simulink model "Resorte_Amoritguador"  (R2025a)
settings: Solver=VariableStepAuto  StartTime=0.0  StopTime=100  RelTol=1e-8
undefined symbols (not defined in the file): gamma, k, m
libraries: fl_lib x6, nesl_utility x3, sdl_lib x1
settings Model: Creator=LAPTOP  LastModifiedBy=LAPTOP

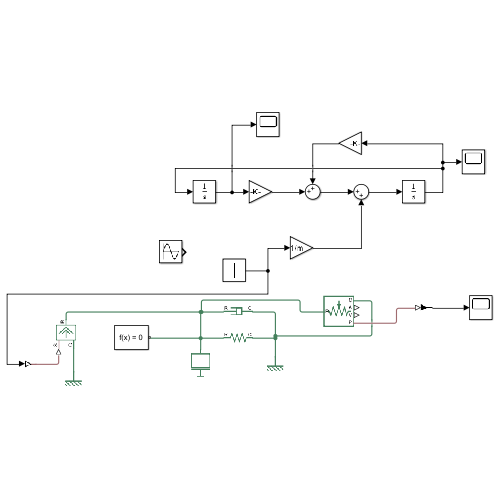
[thumbnail: Simulink's stored preview of the top-level diagram]
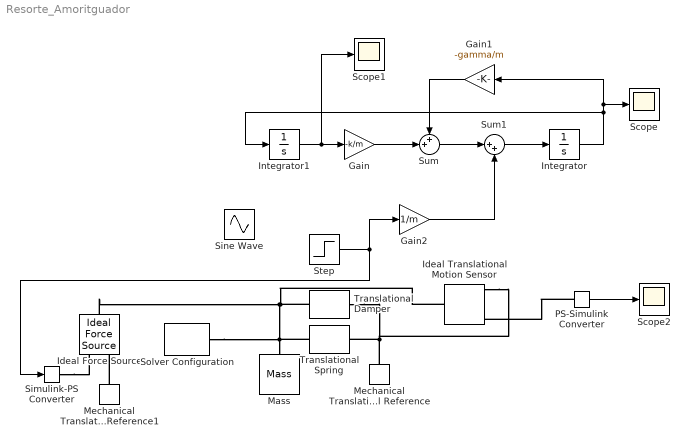
== system Resorte_Amoritguador ==
  Gain : Gain  Gain=-k/m
  Gain1 : Gain  Gain=-gamma/m
  Gain2 : Gain  Gain=1/m
  Ideal Force Source : fl_lib/Mechanical/Mechanical Sources/Ideal Force Source
  Ideal Translational Motion Sensor : fl_lib/Mechanical/Mechanical Sensors/Ideal Translational Motion Sensor  reference=foundation.enum.MeasurementReference.difference  acceleration_port=true  velocity_port=true  position_port=true  offset=0 m
      settings: InternalSimscapePortConfiguration="{\"Bottom\":[],\"Left\":[{\"id\":\"R\",\"label\":\"R\",\"type\":\"foundation.mechanical.translational.translational\"}],\"Right\":[{\"id\":\"C\",\"label\":\"C\",\"type\":\"foundation.mechanical.translational.translational\"},{\"id\":\"A\",\"label\":\"A\",\"type\":\"output\"},{\"id\":\"V\",\"label\":\"V\",\"type\":\"output\"},{\"id\":\"P\",\"label\":\"P\",\"type\":\"output\"}],\"Top\":[]}"
  Integrator : Integrator  InitialCondition=1
  Integrator1 : Integrator
  Mass : fl_lib/Mechanical/Translational Elements/Mass  mass=1 kg  num_ports=foundation.enum.numPorts2.one  v_specify=off  v_priority=High  v=0 m/s  v_nominal_specify=off  v_nominal_value=1  v_nominal_unit=m/s  f_specify=off  f_priority=None  f=0 N  f_nominal_specify=off  f_nominal_value=1  f_nominal_unit=N
  Mechanical Translational Reference : fl_lib/Mechanical/Translational Elements/Mechanical Translational Reference
  Mechanical Translational Reference1 : fl_lib/Mechanical/Translational Elements/Mechanical Translational Reference
  PS-Simulink Converter : nesl_utility/PS-Simulink Converter  PhysicalDomain=network_engine_domain  SubClassName=ps_output  LeftPortType=input  RightPortType=output  PseudoPeriodic=off  Frequencies=[]  VectorFormat=inherit  Unit=mm  AffineConversion=off
  Scope : Scope
      settings: ActiveDisplayYMinimum=-0.99836640803598919  ActiveDisplayYMaximum=1.2220407120039987
  Scope1 : Scope
      settings: ActiveDisplayYMinimum=-0.45113896464501263  ActiveDisplayYMaximum=0.66712367458581923
  Scope2 : Scope
      settings: ActiveDisplayYMinimum=-0.14841442149301454  ActiveDisplayYMaximum=1.1640855785069844  DataLoggingVariableName=ScopeData2
  Simulink-PS Converter : nesl_utility/Simulink-PS Converter  PhysicalDomain=network_engine_domain  SubClassName=ps_input  LeftPortType=input  RightPortType=output  PseudoPeriodic=off  Frequencies=[]  NoiseDistribution=none  NoiseParameters=[]  Unit=1  AffineConversion=off  FilteringAndDerivatives=provide  SimscapeFilterOrder=1  InputFilterTimeConstant=0.001  UdotUserProvided=0
  Sine Wave : Sin  SampleTime=0
  Solver Configuration : nesl_utility/Solver Configuration  PhysicalDomain=network_engine_domain  SubClassName=solver  LeftPortType=input  RightPortType=generic  Tones=[]  Harmonics=[]  SimulateNoise=off  Profile=off  UseLocalSampling=off  EnableSwitchedLinearOptims=on  FrequencyDomain=off  UseCCode=off  RelTol=0.001  AbsTol=0.001  MinStep=1e-09  ToWorkspace=off  RevertToSquareIcSolve=off  NumHomotopyIterations=100  PhasorMode=off  PhasorModeNumHarmonics=1  ConsistencySolver=NEWTON_XTOL_AFTER_FTOL  IndexReductionMethod=DerivativeReplacement  DoDC=off  ResidualTolerance=1e-09  ConsistencyTolSource=GLOBAL  ConsistencyAbsTol=0.001  ConsistencyRelTol=0.001  ConsistencyTolFactor=0.001  UseLocalSolver=off  LocalSolverChoice=NE_BACKWARD_EULER_ADVANCER  ResolveIndetEquations=on  FunctionEvalNumThread=1  LocalSolverSampleTime=0.001  DoFixedCost=off  MaxNonlinIter=3  MaxModeIter=2  ComputeImpulses=off  ImpulseIterations=2  LinearAlgebra=auto  LinearAlgebraNumThread=0  EquationFormulation=NE_TIME_EF  DelaysMemoryBudget=1024  AutomaticFiltering=on  FilteringTimeConstant=0.001  PartitionStorageMethod=AS_NEEDED  PartitionMemoryBudget=1024  PartitionMethod=ROBUST  MultibodyUseLocalSolver=off  MultibodyLocalSolverChoice=ODE1  MultibodyLocalSolverSampleTime=0.001
  Step : Step  SampleTime=0
  Sum : Sum  Inputs=++|
  Sum1 : Sum  Inputs=|++
  Translational Damper : sdl_lib/Couplings & Drives/Springs & Dampers/Translational Damper  D=100 N*s/m  thermal_port=simscape.enum.thermaleffects.omit  thermal_mass=50 kJ/K  temperature_specify=off  temperature_priority=High  temperature=300 K  temperature_nominal_specify=off  temperature_nominal_value=1  temperature_nominal_unit=K
  Translational Spring : fl_lib/Mechanical/Translational Elements/Translational Spring  spr_rate=1000 N/m  v_specify=off  v_priority=None  v=0 m/s  v_nominal_specify=off  v_nominal_value=1  v_nominal_unit=m/s  f_specify=off  f_priority=None  f=0 N  f_nominal_specify=off  f_nominal_value=1  f_nominal_unit=N  x_specify=off  x_priority=High  x=0 m  x_nominal_specify=off  x_nominal_value=1  x_nominal_unit=m
  wires:
  Sum/1 -> Sum1/1
  Sum1/1 -> Integrator/1
  Integrator1/1 -> Scope1/1, Gain/1
  Gain/1 -> Sum/2
  Integrator/1 -> Scope/1, Gain1/1, Integrator1/1
  Gain1/1 -> Sum/1
  Gain2/1 -> Sum1/2
  Step/1 -> Simulink-PS Converter/1, Gain2/1
  PS-Simulink Converter/1 -> Scope2/1
  connections:
  Mechanical Translational Reference/LConn1 -- Ideal Translational Motion Sensor/RConn1 -- Translational Damper/RConn1 -- Translational Spring/RConn1
  Translational Damper/LConn1 -- Ideal Translational Motion Sensor/LConn1 -- Ideal Force Source/LConn1 -- Solver Configuration/RConn1 -- Translational Spring/LConn1 -- Mass/LConn1
  Mechanical Translational Reference1/LConn1 -- Ideal Force Source/RConn2
  Simulink-PS Converter/RConn1 -- Ideal Force Source/RConn1
  PS-Simulink Converter/LConn1 -- Ideal Translational Motion Sensor/RConn4
